simulink model "Landing_Gear_Simscape_multibody"  (R2026a)
settings: Solver=ode15s  StopTime=4.5  MaxStep=0.001  AbsTol=1e-3  EnableMultiTasking=on
libraries: sm_lib x42, nesl_utility x10, simulink x1
settings Model: Creator=USER  LastModifiedBy=USER
settings DebuggingCC: SubsystemReferenceDiagnosticForUnitTest=warning
settings SimscapeCC: SimscapeNominalValues="[{\"value\":\"1\",\"unit\":\"A\"},{\"value\":\"1\",\"unit\":\"bar\"},{\"value\":\"1\",\"unit\":\"cm^2\"},{\"value\":\"1\",\"unit\":\"cm^3/s\"},{\"value\":\"1\",\"unit\":\"kJ/kg\"},{\"value\":\"1\",\"unit\":\"kW\"},{\"value\":\"1\",\"unit\":\"l\"},{\"value\":\"1\",\"unit\":\"N\"},{\"value\":\"1\",\"unit\":\"N*m\"},{\"value\":\"1\",\"unit\":\"V\"}]"

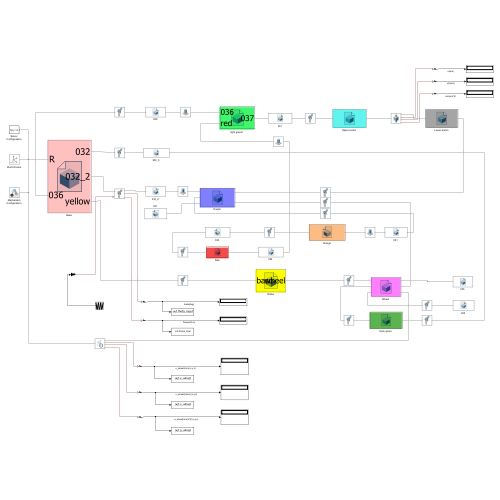
[thumbnail: Simulink's stored preview of the top-level diagram]
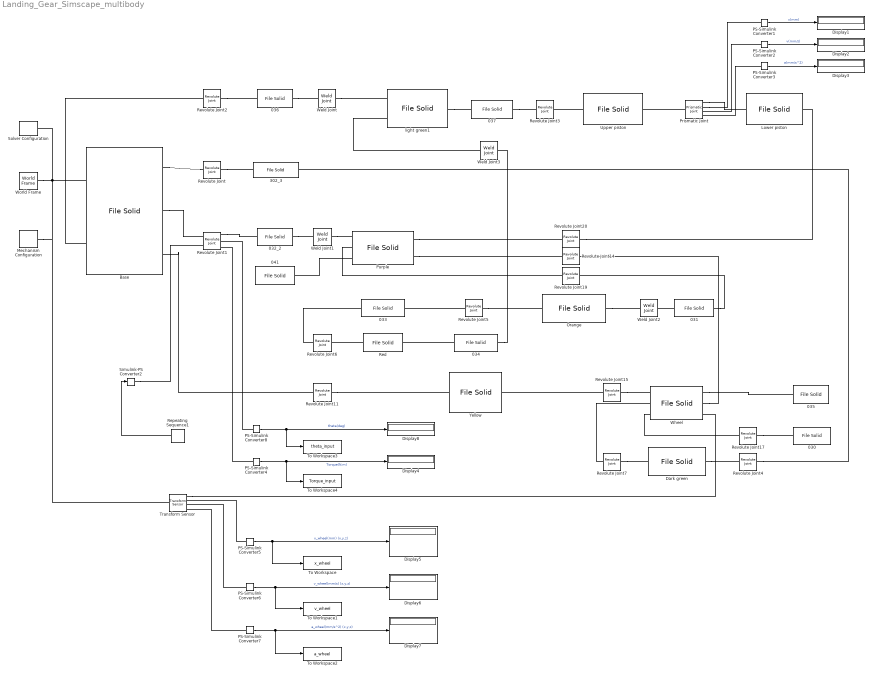
== system Landing_Gear_Simscape_multibody ==
  030 : sm_lib/Body Elements/File Solid  ExtGeomFileName=C:\Users\USER\Desktop\Term project Machinary\Term-Project-2103322-Design-of-Mechanism_Landing_Gear_Mechanism\simulation\cad\Parts\D0493-030.step  UnitType=FromFile  ExtGeomFileUnits=m  StepReaderType=HEX  ExportConvexHullGeometry=off  InertiaType=CalculateFromGeometry  BasedOnType=Density  Density=1000  DensityUnits=kg/m^3  Mass=1  MassUnits=kg  CenterOfMass=[0 0 0]  CenterOfMassUnits=m  MomentsOfInertia=[1 1 1]  MomentsOfInertiaUnits=kg*m^2  ProductsOfInertia=[0 0 0]  ProductsOfInertiaUnits=kg*m^2  GraphicType=FromGeometry  MarkerShape=Sphere  MarkerSize=10  GraphicVisPropType=FromFileVisualProperties  GraphicDiffuseColor=[0.5 0.5 0.5]  GraphicOpacity=1  GraphicSpecularColor=[0.5 0.5 0.5 1.0]  GraphicAmbientColor=[0.15 0.15 0.15 1.0]  GraphicEmissiveColor=[0.0 0.0 0.0 1.0]  GraphicShininess=75  DoExposeReferenceFrame=off  SerializedFrames=|
      | <Frames>
      | 
      |   <Frame>
      |     <Id>Frame1</Id>
      |     <Value>
      |       <Name>wheel</Name>
      |       <Origin>
      |         <Source>GeometricFeature</Source>
      |         <FeatureName>planar surface 2</FeatureName>
      |       </Origin>
      |       <PrimaryAxis>
      |         <DefinedDirection>+Z</DefinedDirection>
      |         <Source>ReferenceFrame</Source>
      |         <SourceDirection>+Z</SourceDirection>
      |         <FeatureName></FeatureName>
      |       </PrimaryAxis>
      |       <SecondaryAxis>
      |         <DefinedDirection>+X</DefinedDirection>
      |         <Source>ReferenceFrame</Source>
      |         <SourceDirection>+X</SourceDirection>
      |         <FeatureName></FeatureName>
      |       </SecondaryAxis>
      |     </Value>
      |   </Frame>
      | 
      | </Frames>
  031 : sm_lib/Body Elements/File Solid  ExtGeomFileName=C:\Users\USER\Desktop\Term project Machinary\Term-Project-2103322-Design-of-Mechanism_Landing_Gear_Mechanism\simulation\cad\Parts\D0493-031.step  UnitType=FromFile  ExtGeomFileUnits=m  StepReaderType=HEX  ExportConvexHullGeometry=off  InertiaType=CalculateFromGeometry  BasedOnType=Density  Density=1000  DensityUnits=kg/m^3  Mass=1  MassUnits=kg  CenterOfMass=[0 0 0]  CenterOfMassUnits=m  MomentsOfInertia=[1 1 1]  MomentsOfInertiaUnits=kg*m^2  ProductsOfInertia=[0 0 0]  ProductsOfInertiaUnits=kg*m^2  GraphicType=FromGeometry  MarkerShape=Sphere  MarkerSize=10  GraphicVisPropType=FromFileVisualProperties  GraphicDiffuseColor=[0.5 0.5 0.5]  GraphicOpacity=1  GraphicSpecularColor=[0.5 0.5 0.5 1.0]  GraphicAmbientColor=[0.15 0.15 0.15 1.0]  GraphicEmissiveColor=[0.0 0.0 0.0 1.0]  GraphicShininess=75  DoExposeReferenceFrame=off  SerializedFrames=|
      | <Frames>
      | 
      |   <Frame>
      |     <Id>Frame1</Id>
      |     <Value>
      |       <Name>orange</Name>
      |       <Origin>
      |         <Source>GeometricFeature</Source>
      |         <FeatureName>planar surface 1</FeatureName>
      |       </Origin>
      |       <PrimaryAxis>
      |         <DefinedDirection>+Z</DefinedDirection>
      |         <Source>ReferenceFrame</Source>
      |         <SourceDirection>+Z</SourceDirection>
      |         <FeatureName></FeatureName>
      |       </PrimaryAxis>
      |       <SecondaryAxis>
      |         <DefinedDirection>+X</DefinedDirection>
      |         <Source>ReferenceFrame</Source>
      |         <SourceDirection>+X</SourceDirection>
      |         <FeatureName></FeatureName>
      |       </SecondaryAxis>
      |     </Value>
      |   </Frame>
      | 
      |   <Frame>
      |     <Id>Frame2</Id>
      |     <Value>
      |       <Name>purple</Name>
      |       <Origin>
      |         <Source>GeometricFeature</Source>
      |         <FeatureName>cylindrical surface 2</FeatureName>
      |       </Origin>
      |       <PrimaryAxis>
      |         <DefinedDirection>+Z</DefinedDirection>
      |         <Source>ReferenceFrame</Source>
      |         <SourceDirection>+Z</SourceDirection>
      |         <FeatureName></FeatureName>
      |       </PrimaryAxis>
      |       <SecondaryAxis>
      |         <DefinedDirection>+X</DefinedDirection>
      |         <Source>ReferenceFrame</Source>
      |         <SourceDirection>+X</SourceDirection>
      |         <FeatureName></FeatureName>
      |       </SecondaryAxis>
      |     </Value>
      |   </Frame>
      | 
      | </Frames>
  032_2 : sm_lib/Body Elements/File Solid  ExtGeomFileName=C:\Users\USER\Desktop\Term project Machinary\Term-Project-2103322-Design-of-Mechanism_Landing_Gear_Mechanism\simulation\cad\Parts\D0493-032_2.step  UnitType=FromFile  ExtGeomFileUnits=m  StepReaderType=HEX  ExportConvexHullGeometry=off  InertiaType=CalculateFromGeometry  BasedOnType=Density  Density=1000  DensityUnits=kg/m^3  Mass=1  MassUnits=kg  CenterOfMass=[0 0 0]  CenterOfMassUnits=m  MomentsOfInertia=[1 1 1]  MomentsOfInertiaUnits=kg*m^2  ProductsOfInertia=[0 0 0]  ProductsOfInertiaUnits=kg*m^2  GraphicType=FromGeometry  MarkerShape=Sphere  MarkerSize=10  GraphicVisPropType=FromFileVisualProperties  GraphicDiffuseColor=[0.5 0.5 0.5]  GraphicOpacity=1  GraphicSpecularColor=[0.5 0.5 0.5 1.0]  GraphicAmbientColor=[0.15 0.15 0.15 1.0]  GraphicEmissiveColor=[0.0 0.0 0.0 1.0]  GraphicShininess=75  DoExposeReferenceFrame=off  SerializedFrames=|
      | <Frames>
      | 
      |   <Frame>
      |     <Id>Frame1</Id>
      |     <Value>
      |       <Name>base</Name>
      |       <Origin>
      |         <Source>GeometricFeature</Source>
      |         <FeatureName>planar surface 1</FeatureName>
      |       </Origin>
      |       <PrimaryAxis>
      |         <DefinedDirection>+Z</DefinedDirection>
      |         <Source>ReferenceFrame</Source>
      |         <SourceDirection>+Z</SourceDirection>
      |         <FeatureName></FeatureName>
      |       </PrimaryAxis>
      |       <SecondaryAxis>
      |         <DefinedDirection>+X</DefinedDirection>
      |         <Source>ReferenceFrame</Source>
      |         <SourceDirection>+X</SourceDirection>
      |         <FeatureName></FeatureName>
      |       </SecondaryAxis>
      |     </Value>
      |   </Frame>
      | 
      |   <Frame>
      |     <Id>Frame2</Id>
      |     <Value>
      |       <Name>purple</Name>
      |       <Origin>
      |         <Source>GeometricFeature</Source>
      |         <FeatureName>cylindrical surface 2</FeatureName>
      |       </Origin>
      |       <PrimaryAxis>
      |         <DefinedDirection>+Z</DefinedDirection>
      |         <Source>ReferenceFrame</Source>
      |         <SourceDirection>+Z</SourceDirection>
      |         <FeatureName></FeatureName>
      |       </PrimaryAxis>
      |       <SecondaryAxis>
      |         <DefinedDirection>+X</DefinedDirection>
      |         <Source>ReferenceFrame</Source>
      |         <SourceDirection>+X</SourceDirection>
      |         <FeatureName></FeatureName>
      |       </SecondaryAxis>
      |     </Value>
      |   </Frame>
      | 
      | </Frames>
  033 : sm_lib/Body Elements/File Solid  ExtGeomFileName=C:\Users\USER\Desktop\Term project Machinary\Term-Project-2103322-Design-of-Mechanism_Landing_Gear_Mechanism\simulation\cad\Parts\D0493-033.step  UnitType=FromFile  ExtGeomFileUnits=m  StepReaderType=HEX  ExportConvexHullGeometry=off  InertiaType=CalculateFromGeometry  BasedOnType=Density  Density=1000  DensityUnits=kg/m^3  Mass=1  MassUnits=kg  CenterOfMass=[0 0 0]  CenterOfMassUnits=m  MomentsOfInertia=[1 1 1]  MomentsOfInertiaUnits=kg*m^2  ProductsOfInertia=[0 0 0]  ProductsOfInertiaUnits=kg*m^2  GraphicType=FromGeometry  MarkerShape=Sphere  MarkerSize=10  GraphicVisPropType=FromFileVisualProperties  GraphicDiffuseColor=[0.5 0.5 0.5]  GraphicOpacity=1  GraphicSpecularColor=[0.5 0.5 0.5 1.0]  GraphicAmbientColor=[0.15 0.15 0.15 1.0]  GraphicEmissiveColor=[0.0 0.0 0.0 1.0]  GraphicShininess=75  DoExposeReferenceFrame=off  SerializedFrames=|
      | <Frames>
      | 
      |   <Frame>
      |     <Id>Frame1</Id>
      |     <Value>
      |       <Name>orange</Name>
      |       <Origin>
      |         <Source>GeometricFeature</Source>
      |         <FeatureName>planar surface 2</FeatureName>
      |       </Origin>
      |       <PrimaryAxis>
      |         <DefinedDirection>+Z</DefinedDirection>
      |         <Source>ReferenceFrame</Source>
      |         <SourceDirection>+Z</SourceDirection>
      |         <FeatureName></FeatureName>
      |       </PrimaryAxis>
      |       <SecondaryAxis>
      |         <DefinedDirection>+X</DefinedDirection>
      |         <Source>ReferenceFrame</Source>
      |         <SourceDirection>+X</SourceDirection>
      |         <FeatureName></FeatureName>
      |       </SecondaryAxis>
      |     </Value>
      |   </Frame>
      | 
      |   <Frame>
      |     <Id>Frame2</Id>
      |     <Value>
      |       <Name>red</Name>
      |       <Origin>
      |         <Source>GeometricFeature</Source>
      |         <FeatureName>cylindrical surface 2</FeatureName>
      |       </Origin>
      |       <PrimaryAxis>
      |         <DefinedDirection>+Z</DefinedDirection>
      |         <Source>ReferenceFrame</Source>
      |         <SourceDirection>+Z</SourceDirection>
      |         <FeatureName></FeatureName>
      |       </PrimaryAxis>
      |       <SecondaryAxis>
      |         <DefinedDirection>+X</DefinedDirection>
      |         <Source>ReferenceFrame</Source>
      |         <SourceDirection>+X</SourceDirection>
      |         <FeatureName></FeatureName>
      |       </SecondaryAxis>
      |     </Value>
      |   </Frame>
      | 
      | </Frames>
  034 : sm_lib/Body Elements/File Solid  ExtGeomFileName=C:\Users\USER\Desktop\Term project Machinary\Term-Project-2103322-Design-of-Mechanism_Landing_Gear_Mechanism\simulation\cad\Parts\D0493-034.step  UnitType=FromFile  ExtGeomFileUnits=m  StepReaderType=HEX  ExportConvexHullGeometry=off  InertiaType=CalculateFromGeometry  BasedOnType=Density  Density=1000  DensityUnits=kg/m^3  Mass=1  MassUnits=kg  CenterOfMass=[0 0 0]  CenterOfMassUnits=m  MomentsOfInertia=[1 1 1]  MomentsOfInertiaUnits=kg*m^2  ProductsOfInertia=[0 0 0]  ProductsOfInertiaUnits=kg*m^2  GraphicType=FromGeometry  MarkerShape=Sphere  MarkerSize=10  GraphicVisPropType=FromFileVisualProperties  GraphicDiffuseColor=[0.5 0.5 0.5]  GraphicOpacity=1  GraphicSpecularColor=[0.5 0.5 0.5 1.0]  GraphicAmbientColor=[0.15 0.15 0.15 1.0]  GraphicEmissiveColor=[0.0 0.0 0.0 1.0]  GraphicShininess=75  DoExposeReferenceFrame=off  SerializedFrames=|
      | <Frames>
      | 
      |   <Frame>
      |     <Id>Frame1</Id>
      |     <Value>
      |       <Name>red</Name>
      |       <Origin>
      |         <Source>GeometricFeature</Source>
      |         <FeatureName>planar surface 2</FeatureName>
      |       </Origin>
      |       <PrimaryAxis>
      |         <DefinedDirection>+Z</DefinedDirection>
      |         <Source>ReferenceFrame</Source>
      |         <SourceDirection>+Z</SourceDirection>
      |         <FeatureName></FeatureName>
      |       </PrimaryAxis>
      |       <SecondaryAxis>
      |         <DefinedDirection>+X</DefinedDirection>
      |         <Source>ReferenceFrame</Source>
      |         <SourceDirection>+X</SourceDirection>
      |         <FeatureName></FeatureName>
      |       </SecondaryAxis>
      |     </Value>
      |   </Frame>
      | 
      |   <Frame>
      |     <Id>Frame2</Id>
      |     <Value>
      |       <Name>lg</Name>
      |       <Origin>
      |         <Source>GeometricFeature</Source>
      |         <FeatureName>planar surface 2</FeatureName>
      |       </Origin>
      |       <PrimaryAxis>
      |         <DefinedDirection>+Z</DefinedDirection>
      |         <Source>ReferenceFrame</Source>
      |         <SourceDirection>+Z</SourceDirection>
      |         <FeatureName></FeatureName>
      |       </PrimaryAxis>
      |       <SecondaryAxis>
      |         <DefinedDirection>+X</DefinedDirection>
      |         <Source>ReferenceFrame</Source>
      |         <SourceDirection>+X</SourceDirection>
      |         <FeatureName></FeatureName>
      |       </SecondaryAxis>
      |     </Value>
      |   </Frame>
      | 
      | </Frames>
  035 : sm_lib/Body Elements/File Solid  ExtGeomFileName=C:\Users\USER\Desktop\Term project Machinary\Term-Project-2103322-Design-of-Mechanism_Landing_Gear_Mechanism\simulation\cad\Parts\D0493-035.step  UnitType=FromFile  ExtGeomFileUnits=m  StepReaderType=HEX  ExportConvexHullGeometry=off  InertiaType=CalculateFromGeometry  BasedOnType=Density  Density=1000  DensityUnits=kg/m^3  Mass=1  MassUnits=kg  CenterOfMass=[0 0 0]  CenterOfMassUnits=m  MomentsOfInertia=[1 1 1]  MomentsOfInertiaUnits=kg*m^2  ProductsOfInertia=[0 0 0]  ProductsOfInertiaUnits=kg*m^2  GraphicType=FromGeometry  MarkerShape=Sphere  MarkerSize=10  GraphicVisPropType=FromFileVisualProperties  GraphicDiffuseColor=[0.5 0.5 0.5]  GraphicOpacity=1  GraphicSpecularColor=[0.5 0.5 0.5 1.0]  GraphicAmbientColor=[0.15 0.15 0.15 1.0]  GraphicEmissiveColor=[0.0 0.0 0.0 1.0]  GraphicShininess=75  DoExposeReferenceFrame=off  SerializedFrames=|
      | <Frames>
      | 
      |   <Frame>
      |     <Id>Frame1</Id>
      |     <Value>
      |       <Name>wheel</Name>
      |       <Origin>
      |         <Source>GeometricFeature</Source>
      |         <FeatureName>planar surface 2</FeatureName>
      |       </Origin>
      |       <PrimaryAxis>
      |         <DefinedDirection>+Z</DefinedDirection>
      |         <Source>ReferenceFrame</Source>
      |         <SourceDirection>+Z</SourceDirection>
      |         <FeatureName></FeatureName>
      |       </PrimaryAxis>
      |       <SecondaryAxis>
      |         <DefinedDirection>+X</DefinedDirection>
      |         <Source>ReferenceFrame</Source>
      |         <SourceDirection>+X</SourceDirection>
      |         <FeatureName></FeatureName>
      |       </SecondaryAxis>
      |     </Value>
      |   </Frame>
      | 
      | </Frames>
  036 : sm_lib/Body Elements/File Solid  ExtGeomFileName=C:\Users\USER\Desktop\Term project Machinary\Term-Project-2103322-Design-of-Mechanism_Landing_Gear_Mechanism\simulation\cad\Parts\D0493-036.step  UnitType=FromFile  ExtGeomFileUnits=m  StepReaderType=HEX  ExportConvexHullGeometry=off  InertiaType=CalculateFromGeometry  BasedOnType=Density  Density=1000  DensityUnits=kg/m^3  Mass=1  MassUnits=kg  CenterOfMass=[0 0 0]  CenterOfMassUnits=m  MomentsOfInertia=[1 1 1]  MomentsOfInertiaUnits=kg*m^2  ProductsOfInertia=[0 0 0]  ProductsOfInertiaUnits=kg*m^2  GraphicType=FromGeometry  MarkerShape=Sphere  MarkerSize=10  GraphicVisPropType=FromFileVisualProperties  GraphicDiffuseColor=[0.5 0.5 0.5]  GraphicOpacity=1  GraphicSpecularColor=[0.5 0.5 0.5 1.0]  GraphicAmbientColor=[0.15 0.15 0.15 1.0]  GraphicEmissiveColor=[0.0 0.0 0.0 1.0]  GraphicShininess=75  DoExposeReferenceFrame=off  SerializedFrames=|
      | <Frames>
      | 
      |   <Frame>
      |     <Id>Frame1</Id>
      |     <Value>
      |       <Name>base</Name>
      |       <Origin>
      |         <Source>GeometricFeature</Source>
      |         <FeatureName>planar surface 2</FeatureName>
      |       </Origin>
      |       <PrimaryAxis>
      |         <DefinedDirection>+Z</DefinedDirection>
      |         <Source>ReferenceFrame</Source>
      |         <SourceDirection>+Z</SourceDirection>
      |         <FeatureName></FeatureName>
      |       </PrimaryAxis>
      |       <SecondaryAxis>
      |         <DefinedDirection>+X</DefinedDirection>
      |         <Source>ReferenceFrame</Source>
      |         <SourceDirection>+X</SourceDirection>
      |         <FeatureName></FeatureName>
      |       </SecondaryAxis>
      |     </Value>
      |   </Frame>
      | 
      |   <Frame>
      |     <Id>Frame2</Id>
      |     <Value>
      |       <Name>light g</Name>
      |       <Origin>
      |         <Source>GeometricFeature</Source>
      |         <FeatureName>cylindrical surface 2</FeatureName>
      |       </Origin>
      |       <PrimaryAxis>
      |         <DefinedDirection>+Z</DefinedDirection>
      |         <Source>ReferenceFrame</Source>
      |         <SourceDirection>+Z</SourceDirection>
      |         <FeatureName></FeatureName>
      |       </PrimaryAxis>
      |       <SecondaryAxis>
      |         <DefinedDirection>+X</DefinedDirection>
      |         <Source>ReferenceFrame</Source>
      |         <SourceDirection>+X</SourceDirection>
      |         <FeatureName></FeatureName>
      |       </SecondaryAxis>
      |     </Value>
      |   </Frame>
      | 
      | </Frames>
  037 : sm_lib/Body Elements/File Solid  ExtGeomFileName=C:\Users\USER\Desktop\Term project Machinary\Term-Project-2103322-Design-of-Mechanism_Landing_Gear_Mechanism\simulation\cad\Parts\D0493-037.step  UnitType=FromFile  ExtGeomFileUnits=m  StepReaderType=HEX  ExportConvexHullGeometry=off  InertiaType=CalculateFromGeometry  BasedOnType=Density  Density=1000  DensityUnits=kg/m^3  Mass=1  MassUnits=kg  CenterOfMass=[0 0 0]  CenterOfMassUnits=m  MomentsOfInertia=[1 1 1]  MomentsOfInertiaUnits=kg*m^2  ProductsOfInertia=[0 0 0]  ProductsOfInertiaUnits=kg*m^2  GraphicType=FromGeometry  MarkerShape=Sphere  MarkerSize=10  GraphicVisPropType=FromFileVisualProperties  GraphicDiffuseColor=[0.5 0.5 0.5]  GraphicOpacity=1  GraphicSpecularColor=[0.5 0.5 0.5 1.0]  GraphicAmbientColor=[0.15 0.15 0.15 1.0]  GraphicEmissiveColor=[0.0 0.0 0.0 1.0]  GraphicShininess=75  DoExposeReferenceFrame=off  SerializedFrames=|
      | <Frames>
      | 
      |   <Frame>
      |     <Id>Frame1</Id>
      |     <Value>
      |       <Name>light g</Name>
      |       <Origin>
      |         <Source>GeometricFeature</Source>
      |         <FeatureName>planar surface 1</FeatureName>
      |       </Origin>
      |       <PrimaryAxis>
      |         <DefinedDirection>+Z</DefinedDirection>
      |         <Source>ReferenceFrame</Source>
      |         <SourceDirection>+Z</SourceDirection>
      |         <FeatureName></FeatureName>
      |       </PrimaryAxis>
      |       <SecondaryAxis>
      |         <DefinedDirection>+X</DefinedDirection>
      |         <Source>ReferenceFrame</Source>
      |         <SourceDirection>+X</SourceDirection>
      |         <FeatureName></FeatureName>
      |       </SecondaryAxis>
      |     </Value>
      |   </Frame>
      | 
      |   <Frame>
      |     <Id>Frame2</Id>
      |     <Value>
      |       <Name>upper</Name>
      |       <Origin>
      |         <Source>GeometricFeature</Source>
      |         <FeatureName>circular curve 4</FeatureName>
      |       </Origin>
      |       <PrimaryAxis>
      |         <DefinedDirection>+Z</DefinedDirection>
      |         <Source>ReferenceFrame</Source>
      |         <SourceDirection>+Z</SourceDirection>
      |         <FeatureName></FeatureName>
      |       </PrimaryAxis>
      |       <SecondaryAxis>
      |         <DefinedDirection>+X</DefinedDirection>
      |         <Source>ReferenceFrame</Source>
      |         <SourceDirection>+X</SourceDirection>
      |         <FeatureName></FeatureName>
      |       </SecondaryAxis>
      |     </Value>
      |   </Frame>
      | 
      | </Frames>
  041 : sm_lib/Body Elements/File Solid  ExtGeomFileName=C:\Users\USER\Desktop\Term project Machinary\Term-Project-2103322-Design-of-Mechanism_Landing_Gear_Mechanism\simulation\cad\Parts\D0493-041.step  UnitType=FromFile  ExtGeomFileUnits=m  StepReaderType=HEX  ExportConvexHullGeometry=off  InertiaType=CalculateFromGeometry  BasedOnType=Density  Density=1000  DensityUnits=kg/m^3  Mass=1  MassUnits=kg  CenterOfMass=[0 0 0]  CenterOfMassUnits=m  MomentsOfInertia=[1 1 1]  MomentsOfInertiaUnits=kg*m^2  ProductsOfInertia=[0 0 0]  ProductsOfInertiaUnits=kg*m^2  GraphicType=FromGeometry  MarkerShape=Sphere  MarkerSize=10  GraphicVisPropType=FromFileVisualProperties  GraphicDiffuseColor=[0.5 0.5 0.5]  GraphicOpacity=1  GraphicSpecularColor=[0.5 0.5 0.5 1.0]  GraphicAmbientColor=[0.15 0.15 0.15 1.0]  GraphicEmissiveColor=[0.0 0.0 0.0 1.0]  GraphicShininess=75  DoExposeReferenceFrame=off  SerializedFrames=|
      | <Frames>
      | 
      |   <Frame>
      |     <Id>Frame1</Id>
      |     <Value>
      |       <Name>purple</Name>
      |       <Origin>
      |         <Source>GeometricFeature</Source>
      |         <FeatureName>planar surface 2</FeatureName>
      |       </Origin>
      |       <PrimaryAxis>
      |         <DefinedDirection>+Z</DefinedDirection>
      |         <Source>ReferenceFrame</Source>
      |         <SourceDirection>+Z</SourceDirection>
      |         <FeatureName></FeatureName>
      |       </PrimaryAxis>
      |       <SecondaryAxis>
      |         <DefinedDirection>+X</DefinedDirection>
      |         <Source>ReferenceFrame</Source>
      |         <SourceDirection>+X</SourceDirection>
      |         <FeatureName></FeatureName>
      |       </SecondaryAxis>
      |     </Value>
      |   </Frame>
      | 
      | </Frames>
  302_3 : sm_lib/Body Elements/File Solid  ExtGeomFileName=C:\Users\USER\Desktop\Term project Machinary\Term-Project-2103322-Design-of-Mechanism_Landing_Gear_Mechanism\simulation\cad\Parts\D0493-032_3.step  UnitType=FromFile  ExtGeomFileUnits=m  StepReaderType=HEX  ExportConvexHullGeometry=off  InertiaType=CalculateFromGeometry  BasedOnType=Density  Density=1000  DensityUnits=kg/m^3  Mass=1  MassUnits=kg  CenterOfMass=[0 0 0]  CenterOfMassUnits=m  MomentsOfInertia=[1 1 1]  MomentsOfInertiaUnits=kg*m^2  ProductsOfInertia=[0 0 0]  ProductsOfInertiaUnits=kg*m^2  GraphicType=FromGeometry  MarkerShape=Sphere  MarkerSize=10  GraphicVisPropType=FromFileVisualProperties  GraphicDiffuseColor=[0.5 0.5 0.5]  GraphicOpacity=1  GraphicSpecularColor=[0.5 0.5 0.5 1.0]  GraphicAmbientColor=[0.15 0.15 0.15 1.0]  GraphicEmissiveColor=[0.0 0.0 0.0 1.0]  GraphicShininess=75  DoExposeReferenceFrame=off  SerializedFrames=|
      | <Frames>
      | 
      |   <Frame>
      |     <Id>Frame1</Id>
      |     <Value>
      |       <Name>Base</Name>
      |       <Origin>
      |         <Source>GeometricFeature</Source>
      |         <FeatureName>planar surface 1</FeatureName>
      |       </Origin>
      |       <PrimaryAxis>
      |         <DefinedDirection>+Z</DefinedDirection>
      |         <Source>ReferenceFrame</Source>
      |         <SourceDirection>+Z</SourceDirection>
      |         <FeatureName></FeatureName>
      |       </PrimaryAxis>
      |       <SecondaryAxis>
      |         <DefinedDirection>+X</DefinedDirection>
      |         <Source>ReferenceFrame</Source>
      |         <SourceDirection>+X</SourceDirection>
      |         <FeatureName></FeatureName>
      |       </SecondaryAxis>
      |     </Value>
      |   </Frame>
      | 
      |   <Frame>
      |     <Id>Frame2</Id>
      |     <Value>
      |       <Name>darkgreen</Name>
      |       <Origin>
      |         <Source>GeometricFeature</Source>
      |         <FeatureName>cylindrical surface 1</FeatureName>
      |       </Origin>
      |       <PrimaryAxis>
      |         <DefinedDirection>+Z</DefinedDirection>
      |         <Source>ReferenceFrame</Source>
      |         <SourceDirection>+Z</SourceDirection>
      |         <FeatureName></FeatureName>
      |       </PrimaryAxis>
      |       <SecondaryAxis>
      |         <DefinedDirection>+X</DefinedDirection>
      |         <Source>ReferenceFrame</Source>
      |         <SourceDirection>+X</SourceDirection>
      |         <FeatureName></FeatureName>
      |       </SecondaryAxis>
      |     </Value>
      |   </Frame>
      | 
      | </Frames>
  Base : sm_lib/Body Elements/File Solid  ExtGeomFileName=C:\Users\USER\Desktop\Term project Machinary\Term-Project-2103322-Design-of-Mechanism_Landing_Gear_Mechanism\simulation\cad\Parts\Base.step  UnitType=FromFile  ExtGeomFileUnits=m  StepReaderType=HEX  ExportConvexHullGeometry=off  InertiaType=CalculateFromGeometry  BasedOnType=Density  Density=1000  DensityUnits=kg/m^3  Mass=1  MassUnits=kg  CenterOfMass=[0 0 0]  CenterOfMassUnits=m  MomentsOfInertia=[1 1 1]  MomentsOfInertiaUnits=kg*m^2  ProductsOfInertia=[0 0 0]  ProductsOfInertiaUnits=kg*m^2  GraphicType=FromGeometry  MarkerShape=Sphere  MarkerSize=10  GraphicVisPropType=FromFileVisualProperties  GraphicDiffuseColor=[0.5 0.5 0.5]  GraphicOpacity=1  GraphicSpecularColor=[0.5 0.5 0.5 1.0]  GraphicAmbientColor=[0.15 0.15 0.15 1.0]  GraphicEmissiveColor=[0.0 0.0 0.0 1.0]  GraphicShininess=75  DoExposeReferenceFrame=on  SerializedFrames=|
      | <Frames>
      | 
      |   <Frame>
      |     <Id>Frame1</Id>
      |     <Value>
      |       <Name>032</Name>
      |       <Origin>
      |         <Source>GeometricFeature</Source>
      |         <FeatureName>circular curve 21</FeatureName>
      |       </Origin>
      |       <PrimaryAxis>
      |         <DefinedDirection>+Z</DefinedDirection>
      |         <Source>GeometricFeature</Source>
      |         <SourceDirection>+Z</SourceDirection>
      |         <FeatureName>circular curve 33</FeatureName>
      |       </PrimaryAxis>
      |       <SecondaryAxis>
      |         <DefinedDirection>+Y</DefinedDirection>
      |         <Source>ReferenceFrame</Source>
      |         <SourceDirection>+Y</SourceDirection>
      |         <FeatureName></FeatureName>
      |       </SecondaryAxis>
      |     </Value>
      |   </Frame>
      | 
      |   <Frame>
      |     <Id>Frame2</Id>
      |     <Value>
      |       <Name>032_2</Name>
      |       <Origin>
      |         <Source>GeometricFeature</Source>
      |         <FeatureName>circular curve 35</FeatureName>
      |       </Origin>
      |       <PrimaryAxis>
      |         <DefinedDirection>+Z</DefinedDirection>
      |         <Source>GeometricFeature</Source>
      |         <SourceDirection>+Z</SourceDirection>
      |         <FeatureName>circular curve 35</FeatureName>
      |       </PrimaryAxis>
      |       <SecondaryAxis>
      |         <DefinedDirection>+Y</DefinedDirection>
      |         <Source>ReferenceFrame</Source>
      |         <SourceDirection>+Y</SourceDirection>
      |         <FeatureName></FeatureName>
      |       </SecondaryAxis>
      |     </Value>
      |   </Frame>
      | 
      |   <Frame>
      |     <Id>Frame3</Id>
      |     <Value>
      |       <Name>036</Name>
      |       <Origin>
      |         <Source>GeometricFeature</Source>
      |         <FeatureName>circular curve 89</FeatureName>
      |       </Origin>
      |       <PrimaryAxis>
      |         <DefinedDirection>-Z</DefinedDirection>
      |         <Source>GeometricFeature</Source>
      |         <SourceDirection>+Z</SourceDirection>
      |         <FeatureName>circular curve 89</FeatureName>
      |       </PrimaryAxis>
      |       <SecondaryAxis>
      |         <DefinedDirection>+Y</DefinedDirection>
      |         <Source>ReferenceFrame</Source>
      |         <SourceDirection>+Y</SourceDirection>
      |         <FeatureName></FeatureName>
      |       </SecondaryAxis>
      |     </Value>
      |   </Frame>
      | 
      |   <Frame>
      |     <Id>Frame4</Id>
      |     <Value>
      |       <Name>yellow</Name>
      |       <Origin>
      |         <Source>GeometricFeature</Source>
      |         <FeatureName>circular curve 60</FeatureName>
      |       </Origin>
      |       <PrimaryAxis>
      |         <DefinedDirection>+Z</DefinedDirection>
      |         <Source>GeometricFeature</Source>
      |         <SourceDirection>+Z</SourceDirection>
      |         <FeatureName>circular curve 60</FeatureName>
      |       </PrimaryAxis>
      |       <SecondaryAxis>
      |         <DefinedDirection>+Y</DefinedDirection>
      |         <Source>ReferenceFrame</Source>
      |         <SourceDirection>+Y</SourceDirection>
      |         <FeatureName></FeatureName>
      |       </SecondaryAxis>
      |     </Value>
      |   </Frame>
      | 
      | </Frames>
  Dark green : sm_lib/Body Elements/File Solid  ExtGeomFileName=C:\Users\USER\Desktop\Term project Machinary\Term-Project-2103322-Design-of-Mechanism_Landing_Gear_Mechanism\simulation\cad\Parts\Dark green.step  UnitType=FromFile  ExtGeomFileUnits=m  StepReaderType=HEX  ExportConvexHullGeometry=off  InertiaType=CalculateFromGeometry  BasedOnType=Density  Density=1000  DensityUnits=kg/m^3  Mass=1  MassUnits=kg  CenterOfMass=[0 0 0]  CenterOfMassUnits=m  MomentsOfInertia=[1 1 1]  MomentsOfInertiaUnits=kg*m^2  ProductsOfInertia=[0 0 0]  ProductsOfInertiaUnits=kg*m^2  GraphicType=FromGeometry  MarkerShape=Sphere  MarkerSize=10  GraphicVisPropType=FromFileVisualProperties  GraphicDiffuseColor=[0.5 0.5 0.5]  GraphicOpacity=1  GraphicSpecularColor=[0.5 0.5 0.5 1.0]  GraphicAmbientColor=[0.15 0.15 0.15 1.0]  GraphicEmissiveColor=[0.0 0.0 0.0 1.0]  GraphicShininess=75  DoExposeReferenceFrame=off  SerializedFrames=|
      | <Frames>
      | 
      |   <Frame>
      |     <Id>Frame1</Id>
      |     <Value>
      |       <Name>wheel</Name>
      |       <Origin>
      |         <Source>GeometricFeature</Source>
      |         <FeatureName>circular curve 51</FeatureName>
      |       </Origin>
      |       <PrimaryAxis>
      |         <DefinedDirection>+Z</DefinedDirection>
      |         <Source>GeometricFeature</Source>
      |         <SourceDirection>+Z</SourceDirection>
      |         <FeatureName>circular curve 51</FeatureName>
      |       </PrimaryAxis>
      |       <SecondaryAxis>
      |         <DefinedDirection>+Y</DefinedDirection>
      |         <Source>ReferenceFrame</Source>
      |         <SourceDirection>+Y</SourceDirection>
      |         <FeatureName></FeatureName>
      |       </SecondaryAxis>
      |     </Value>
      |   </Frame>
      | 
      |   <Frame>
      |     <Id>Frame2</Id>
      |     <Value>
      |       <Name>base</Name>
      |       <Origin>
      |         <Source>GeometricFeature</Source>
      |         <FeatureName>cylindrical surface 10</FeatureName>
      |       </Origin>
      |       <PrimaryAxis>
      |         <DefinedDirection>+Z</DefinedDirection>
      |         <Source>GeometricFeature</Source>
      |         <SourceDirection>+Z</SourceDirection>
      |         <FeatureName>cylindrical surface 10</FeatureName>
      |       </PrimaryAxis>
      |       <SecondaryAxis>
      |         <DefinedDirection>+Y</DefinedDirection>
      |         <Source>ReferenceFrame</Source>
      |         <SourceDirection>+Y</SourceDirection>
      |         <FeatureName></FeatureName>
      |       </SecondaryAxis>
      |     </Value>
      |   </Frame>
      | 
      | </Frames>
  Display{1..8} (8 alike) : Display
  Lower piston : sm_lib/Body Elements/File Solid  ExtGeomFileName=C:\Users\USER\Desktop\Term project Machinary\Term-Project-2103322-Design-of-Mechanism_Landing_Gear_Mechanism\simulation\cad\Parts\Lower_Piston2.step  UnitType=FromFile  ExtGeomFileUnits=m  StepReaderType=HEX  ExportConvexHullGeometry=off  InertiaType=CalculateFromGeometry  BasedOnType=Density  Density=1000  DensityUnits=kg/m^3  Mass=1  MassUnits=kg  CenterOfMass=[0 0 0]  CenterOfMassUnits=m  MomentsOfInertia=[1 1 1]  MomentsOfInertiaUnits=kg*m^2  ProductsOfInertia=[0 0 0]  ProductsOfInertiaUnits=kg*m^2  GraphicType=FromGeometry  MarkerShape=Sphere  MarkerSize=10  GraphicVisPropType=FromFileVisualProperties  GraphicDiffuseColor=[0.5 0.5 0.5]  GraphicOpacity=1  GraphicSpecularColor=[0.5 0.5 0.5 1.0]  GraphicAmbientColor=[0.15 0.15 0.15 1.0]  GraphicEmissiveColor=[0.0 0.0 0.0 1.0]  GraphicShininess=75  DoExposeReferenceFrame=off  SerializedFrames=|
      | <Frames>
      | 
      |   <Frame>
      |     <Id>Frame1</Id>
      |     <Value>
      |       <Name>upper</Name>
      |       <Origin>
      |         <Source>GeometricFeature</Source>
      |         <FeatureName>circular curve 40</FeatureName>
      |       </Origin>
      |       <PrimaryAxis>
      |         <DefinedDirection>-Z</DefinedDirection>
      |         <Source>GeometricFeature</Source>
      |         <SourceDirection>+Z</SourceDirection>
      |         <FeatureName>circular curve 40</FeatureName>
      |       </PrimaryAxis>
      |       <SecondaryAxis>
      |         <DefinedDirection>+X</DefinedDirection>
      |         <Source>ReferenceFrame</Source>
      |         <SourceDirection>+X</SourceDirection>
      |         <FeatureName></FeatureName>
      |       </SecondaryAxis>
      |     </Value>
      |   </Frame>
      | 
      |   <Frame>
      |     <Id>Frame2</Id>
      |     <Value>
      |       <Name>purple</Name>
      |       <Origin>
      |         <Source>GeometricFeature</Source>
      |         <FeatureName>circular curve 37</FeatureName>
      |       </Origin>
      |       <PrimaryAxis>
      |         <DefinedDirection>+Z</DefinedDirection>
      |         <Source>GeometricFeature</Source>
      |         <SourceDirection>+Z</SourceDirection>
      |         <FeatureName>circular curve 37</FeatureName>
      |       </PrimaryAxis>
      |       <SecondaryAxis>
      |         <DefinedDirection>+Y</DefinedDirection>
      |         <Source>ReferenceFrame</Source>
      |         <SourceDirection>+Y</SourceDirection>
      |         <FeatureName></FeatureName>
      |       </SecondaryAxis>
      |     </Value>
      |   </Frame>
      | 
      | </Frames>
  Mechanism Configuration : sm_lib/Utilities/Mechanism Configuration  UniformGravity=Constant  GravityVector=[0 0 -9.80665]  GravityVectorUnits=m/s^2  LinearizationDelta=0.001  JointModeTransitionNonlinearIterations=2
  Orange : sm_lib/Body Elements/File Solid  ExtGeomFileName=C:\Users\USER\Desktop\Term project Machinary\Term-Project-2103322-Design-of-Mechanism_Landing_Gear_Mechanism\simulation\cad\Parts\Orange.step  UnitType=FromFile  ExtGeomFileUnits=m  StepReaderType=HEX  ExportConvexHullGeometry=off  InertiaType=CalculateFromGeometry  BasedOnType=Density  Density=1000  DensityUnits=kg/m^3  Mass=1  MassUnits=kg  CenterOfMass=[0 0 0]  CenterOfMassUnits=m  MomentsOfInertia=[1 1 1]  MomentsOfInertiaUnits=kg*m^2  ProductsOfInertia=[0 0 0]  ProductsOfInertiaUnits=kg*m^2  GraphicType=FromGeometry  MarkerShape=Sphere  MarkerSize=10  GraphicVisPropType=FromFileVisualProperties  GraphicDiffuseColor=[0.5 0.5 0.5]  GraphicOpacity=1  GraphicSpecularColor=[0.5 0.5 0.5 1.0]  GraphicAmbientColor=[0.15 0.15 0.15 1.0]  GraphicEmissiveColor=[0.0 0.0 0.0 1.0]  GraphicShininess=75  DoExposeReferenceFrame=off  SerializedFrames=|
      | <Frames>
      | 
      |   <Frame>
      |     <Id>Frame1</Id>
      |     <Value>
      |       <Name>031</Name>
      |       <Origin>
      |         <Source>GeometricFeature</Source>
      |         <FeatureName>circular curve 22</FeatureName>
      |       </Origin>
      |       <PrimaryAxis>
      |         <DefinedDirection>-Z</DefinedDirection>
      |         <Source>GeometricFeature</Source>
      |         <SourceDirection>+Z</SourceDirection>
      |         <FeatureName>circular curve 22</FeatureName>
      |       </PrimaryAxis>
      |       <SecondaryAxis>
      |         <DefinedDirection>+Y</DefinedDirection>
      |         <Source>ReferenceFrame</Source>
      |         <SourceDirection>+Y</SourceDirection>
      |         <FeatureName></FeatureName>
      |       </SecondaryAxis>
      |     </Value>
      |   </Frame>
      | 
      |   <Frame>
      |     <Id>Frame2</Id>
      |     <Value>
      |       <Name>033</Name>
      |       <Origin>
      |         <Source>GeometricFeature</Source>
      |         <FeatureName>circular curve 58</FeatureName>
      |       </Origin>
      |       <PrimaryAxis>
      |         <DefinedDirection>-Z</DefinedDirection>
      |         <Source>GeometricFeature</Source>
      |         <SourceDirection>+Z</SourceDirection>
      |         <FeatureName>circular curve 58</FeatureName>
      |       </PrimaryAxis>
      |       <SecondaryAxis>
      |         <DefinedDirection>+Y</DefinedDirection>
      |         <Source>ReferenceFrame</Source>
      |         <SourceDirection>+Y</SourceDirection>
      |         <FeatureName></FeatureName>
      |       </SecondaryAxis>
      |     </Value>
      |   </Frame>
      | 
      | </Frames>
  PS-Simulink Converter1 : nesl_utility/PS-Simulink Converter  PhysicalDomain=network_engine_domain  SubClassName=ps_output  LeftPortType=input  RightPortType=output  PseudoPeriodic=off  Frequencies=[]  VectorFormat=inherit  Unit=mm  AffineConversion=off
  PS-Simulink Converter2 : nesl_utility/PS-Simulink Converter  PhysicalDomain=network_engine_domain  SubClassName=ps_output  LeftPortType=input  RightPortType=output  PseudoPeriodic=off  Frequencies=[]  VectorFormat=inherit  Unit=mm/s  AffineConversion=off
  PS-Simulink Converter3 : nesl_utility/PS-Simulink Converter  PhysicalDomain=network_engine_domain  SubClassName=ps_output  LeftPortType=input  RightPortType=output  PseudoPeriodic=off  Frequencies=[]  VectorFormat=inherit  Unit=mm/s^2  AffineConversion=off
  PS-Simulink Converter4 : nesl_utility/PS-Simulink Converter  PhysicalDomain=network_engine_domain  SubClassName=ps_output  LeftPortType=input  RightPortType=output  PseudoPeriodic=off  Frequencies=[]  VectorFormat=1-D array  Unit=N*m  AffineConversion=off
  PS-Simulink Converter5 : nesl_utility/PS-Simulink Converter  PhysicalDomain=network_engine_domain  SubClassName=ps_output  LeftPortType=input  RightPortType=output  PseudoPeriodic=off  Frequencies=[]  VectorFormat=inherit  Unit=mm  AffineConversion=off
  PS-Simulink Converter6 : nesl_utility/PS-Simulink Converter  PhysicalDomain=network_engine_domain  SubClassName=ps_output  LeftPortType=input  RightPortType=output  PseudoPeriodic=off  Frequencies=[]  VectorFormat=inherit  Unit=mm/s  AffineConversion=off
  PS-Simulink Converter7 : nesl_utility/PS-Simulink Converter  PhysicalDomain=network_engine_domain  SubClassName=ps_output  LeftPortType=input  RightPortType=output  PseudoPeriodic=off  Frequencies=[]  VectorFormat=inherit  Unit=mm/s^2  AffineConversion=off
  PS-Simulink Converter8 : nesl_utility/PS-Simulink Converter  PhysicalDomain=network_engine_domain  SubClassName=ps_output  LeftPortType=input  RightPortType=output  PseudoPeriodic=off  Frequencies=[]  VectorFormat=1-D array  Unit=deg  AffineConversion=off
  Prismatic Joint : sm_lib/Joints/Prismatic Joint  JointMode=Normal  CompositeWrenchDir=FollowerOnBase  CompositeWrenchFrame=BaseFrame  SenseConstraintForce=off  SenseConstraintTorque=off  SenseTotalForce=off  SenseTotalTorque=off  PositionTargetSpecify=off  PositionTargetPriority=High  PositionTargetValue=0  PositionTargetValueUnits=m  VelocityTargetSpecify=off  VelocityTargetPriority=High  VelocityTargetValue=0  VelocityTargetValueUnits=m/s  EquilibriumPosition=0  EquilibriumPositionUnits=m  SpringStiffness=0  SpringStiffnessUnits=N/m  DampingCoefficient=0  DampingCoefficientUnits=N/(m/s)  LowerLimitSpecify=off  LowerLimitBound=-1  LowerLimitBoundUnits=m  LowerLimitStiffness=1e6  LowerLimitStiffnessUnits=N/m  LowerLimitDamping=1e3  LowerLimitDampingUnits=N/(m/s)  LowerLimitTransitionRegionWidth=1e-4  LowerLimitTransitionRegionWidthUnits=m  UpperLimitSpecify=off  UpperLimitBound=1  UpperLimitBoundUnits=m  UpperLimitStiffness=1e6  UpperLimitStiffnessUnits=N/m  UpperLimitDamping=1e3  UpperLimitDampingUnits=N/(m/s)  UpperLimitTransitionRegionWidth=1e-4  UpperLimitTransitionRegionWidthUnits=m  TorqueActuationMode=NoTorque  MotionActuationMode=ComputedMotion  SensePosition=on  SenseVelocity=on  SenseAcceleration=on  SenseTorqueForce=off  SenseLowerLimitTorqueForce=off  SenseUpperLimitTorqueForce=off
  Purple : sm_lib/Body Elements/File Solid  ExtGeomFileName=C:\Users\USER\Desktop\Term project Machinary\Term-Project-2103322-Design-of-Mechanism_Landing_Gear_Mechanism\simulation\cad\Parts\Purple.step  UnitType=FromFile  ExtGeomFileUnits=m  StepReaderType=HEX  ExportConvexHullGeometry=off  InertiaType=CalculateFromGeometry  BasedOnType=Density  Density=1000  DensityUnits=kg/m^3  Mass=1  MassUnits=kg  CenterOfMass=[0 0 0]  CenterOfMassUnits=m  MomentsOfInertia=[1 1 1]  MomentsOfInertiaUnits=kg*m^2  ProductsOfInertia=[0 0 0]  ProductsOfInertiaUnits=kg*m^2  GraphicType=FromGeometry  MarkerShape=Sphere  MarkerSize=10  GraphicVisPropType=FromFileVisualProperties  GraphicDiffuseColor=[0.5 0.5 0.5]  GraphicOpacity=1  GraphicSpecularColor=[0.5 0.5 0.5 1.0]  GraphicAmbientColor=[0.15 0.15 0.15 1.0]  GraphicEmissiveColor=[0.0 0.0 0.0 1.0]  GraphicShininess=75  DoExposeReferenceFrame=off  SerializedFrames=|
      | <Frames>
      | 
      |   <Frame>
      |     <Id>Frame1</Id>
      |     <Value>
      |       <Name>base</Name>
      |       <Origin>
      |         <Source>GeometricFeature</Source>
      |         <FeatureName>cylindrical surface 21</FeatureName>
      |       </Origin>
      |       <PrimaryAxis>
      |         <DefinedDirection>+Z</DefinedDirection>
      |         <Source>GeometricFeature</Source>
      |         <SourceDirection>+Z</SourceDirection>
      |         <FeatureName>cylindrical surface 21</FeatureName>
      |       </PrimaryAxis>
      |       <SecondaryAxis>
      |         <DefinedDirection>+Y</DefinedDirection>
      |         <Source>ReferenceFrame</Source>
      |         <SourceDirection>+Y</SourceDirection>
      |         <FeatureName></FeatureName>
      |       </SecondaryAxis>
      |     </Value>
      |   </Frame>
      | 
      |   <Frame>
      |     <Id>Frame2</Id>
      |     <Value>
      |       <Name>lower</Name>
      |       <Origin>
      |         <Source>GeometricFeature</Source>
      |         <FeatureName>circular curve 37</FeatureName>
      |       </Origin>
      |       <PrimaryAxis>
      |         <DefinedDirection>-Z</DefinedDirection>
      |         <Source>GeometricFeature</Source>
      |         <SourceDirection>+Z</SourceDirection>
      |         <FeatureName>circular curve 37</FeatureName>
      |       </PrimaryAxis>
      |       <SecondaryAxis>
      |         <DefinedDirection>+Y</DefinedDirection>
      |         <Source>ReferenceFrame</Source>
      |         <SourceDirection>+Y</SourceDirection>
      |         <FeatureName></FeatureName>
      |       </SecondaryAxis>
      |     </Value>
      |   </Frame>
      | 
      |   <Frame>
      |     <Id>Frame3</Id>
      |     <Value>
      |       <Name>orange</Name>
      |       <Origin>
      |         <Source>GeometricFeature</Source>
      |         <FeatureName>cylindrical surface 33</FeatureName>
      |       </Origin>
      |       <PrimaryAxis>
      |         <DefinedDirection>+Z</DefinedDirection>
      |         <Source>GeometricFeature</Source>
      |         <SourceDirection>+Z</SourceDirection>
      |         <FeatureName>cylindrical surface 33</FeatureName>
      |       </PrimaryAxis>
      |       <SecondaryAxis>
      |         <DefinedDirection>+Y</DefinedDirection>
      |         <Source>ReferenceFrame</Source>
      |         <SourceDirection>+Y</SourceDirection>
      |         <FeatureName></FeatureName>
      |       </SecondaryAxis>
      |     </Value>
      |   </Frame>
      | 
      |   <Frame>
      |     <Id>Frame4</Id>
      |     <Value>
      |       <Name>wheel</Name>
      |       <Origin>
      |         <Source>GeometricFeature</Source>
      |         <FeatureName>circular curve 82</FeatureName>
      |       </Origin>
      |       <PrimaryAxis>
      |         <DefinedDirection>+Z</DefinedDirection>
      |         <Source>GeometricFeature</Source>
      |         <SourceDirection>+Z</SourceDirection>
      |         <FeatureName>circular curve 95</FeatureName>
      |       </PrimaryAxis>
      |       <SecondaryAxis>
      |         <DefinedDirection>+Y</DefinedDirection>
      |         <Source>ReferenceFrame</Source>
      |         <SourceDirection>+Y</SourceDirection>
      |         <FeatureName></FeatureName>
      |       </SecondaryAxis>
      |     </Value>
      |   </Frame>
      | 
      |   <Frame>
      |     <Id>Frame5</Id>
      |     <Value>
      |       <Name>041</Name>
      |       <Origin>
      |         <Source>GeometricFeature</Source>
      |         <FeatureName>circular curve 29</FeatureName>
      |       </Origin>
      |       <PrimaryAxis>
      |         <DefinedDirection>+Z</DefinedDirection>
      |         <Source>GeometricFeature</Source>
      |         <SourceDirection>+Z</SourceDirection>
      |         <FeatureName>circular curve 29</FeatureName>
      |       </PrimaryAxis>
      |       <SecondaryAxis>
      |         <DefinedDirection>+Y</DefinedDirection>
      |         <Source>ReferenceFrame</Source>
      |         <SourceDirection>+Y</SourceDirection>
      |         <FeatureName></FeatureName>
      |       </SecondaryAxis>
      |     </Value>
      |   </Frame>
      | 
      | </Frames>
  Red : sm_lib/Body Elements/File Solid  ExtGeomFileName=C:\Users\USER\Desktop\Term project Machinary\Term-Project-2103322-Design-of-Mechanism_Landing_Gear_Mechanism\simulation\cad\Parts\Red.step  UnitType=FromFile  ExtGeomFileUnits=m  StepReaderType=HEX  ExportConvexHullGeometry=off  InertiaType=CalculateFromGeometry  BasedOnType=Density  Density=1000  DensityUnits=kg/m^3  Mass=1  MassUnits=kg  CenterOfMass=[0 0 0]  CenterOfMassUnits=m  MomentsOfInertia=[1 1 1]  MomentsOfInertiaUnits=kg*m^2  ProductsOfInertia=[0 0 0]  ProductsOfInertiaUnits=kg*m^2  GraphicType=FromGeometry  MarkerShape=Sphere  MarkerSize=10  GraphicVisPropType=FromFileVisualProperties  GraphicDiffuseColor=[0.5 0.5 0.5]  GraphicOpacity=1  GraphicSpecularColor=[0.5 0.5 0.5 1.0]  GraphicAmbientColor=[0.15 0.15 0.15 1.0]  GraphicEmissiveColor=[0.0 0.0 0.0 1.0]  GraphicShininess=75  DoExposeReferenceFrame=off  SerializedFrames=|
      | <Frames>
      | 
      |   <Frame>
      |     <Id>Frame1</Id>
      |     <Value>
      |       <Name>033</Name>
      |       <Origin>
      |         <Source>GeometricFeature</Source>
      |         <FeatureName>cylindrical surface 13</FeatureName>
      |       </Origin>
      |       <PrimaryAxis>
      |         <DefinedDirection>-Z</DefinedDirection>
      |         <Source>GeometricFeature</Source>
      |         <SourceDirection>+Z</SourceDirection>
      |         <FeatureName>cylindrical surface 13</FeatureName>
      |       </PrimaryAxis>
      |       <SecondaryAxis>
      |         <DefinedDirection>+Y</DefinedDirection>
      |         <Source>ReferenceFrame</Source>
      |         <SourceDirection>+Y</SourceDirection>
      |         <FeatureName></FeatureName>
      |       </SecondaryAxis>
      |     </Value>
      |   </Frame>
      | 
      |   <Frame>
      |     <Id>Frame2</Id>
      |     <Value>
      |       <Name>034</Name>
      |       <Origin>
      |         <Source>GeometricFeature</Source>
      |         <FeatureName>circular curve 4</FeatureName>
      |       </Origin>
      |       <PrimaryAxis>
      |         <DefinedDirection>+Z</DefinedDirection>
      |         <Source>GeometricFeature</Source>
      |         <SourceDirection>+Z</SourceDirection>
      |         <FeatureName>circular curve 4</FeatureName>
      |       </PrimaryAxis>
      |       <SecondaryAxis>
      |         <DefinedDirection>+X</DefinedDirection>
      |         <Source>ReferenceFrame</Source>
      |         <SourceDirection>+X</SourceDirection>
      |         <FeatureName></FeatureName>
      |       </SecondaryAxis>
      |     </Value>
      |   </Frame>
      | 
      | </Frames>
  Repeating Sequence1 : simulink/Sources/Repeating Sequence  rep_seq_t=[0 4.5 6 12]  rep_seq_y=[-0.11454782472119 -1.7280948939871 -1.7280948939871 -0.11454782472119]
  Revolute Joint{,2..7,14..15,17,19} (11 alike) : sm_lib/Joints/Revolute Joint  JointMode=Normal  CompositeWrenchDir=FollowerOnBase  CompositeWrenchFrame=BaseFrame  SenseConstraintForce=off  SenseConstraintTorque=off  SenseTotalForce=off  SenseTotalTorque=off  PositionTargetSpecify=off  PositionTargetPriority=High  PositionTargetValue=0  PositionTargetValueUnits=deg  VelocityTargetSpecify=off  VelocityTargetPriority=High  VelocityTargetValue=0  VelocityTargetValueUnits=deg/s  EquilibriumPosition=0  EquilibriumPositionUnits=deg  SpringStiffness=0  SpringStiffnessUnits=N*m/deg  DampingCoefficient=0  DampingCoefficientUnits=N*m/(deg/s)  LowerLimitSpecify=off  LowerLimitBound=-90  LowerLimitBoundUnits=deg  LowerLimitStiffness=1e4  LowerLimitStiffnessUnits=N*m/deg  LowerLimitDamping=10  LowerLimitDampingUnits=N*m/(deg/s)  LowerLimitTransitionRegionWidth=0.1  LowerLimitTransitionRegionWidthUnits=deg  UpperLimitSpecify=off  UpperLimitBound=90  UpperLimitBoundUnits=deg  UpperLimitStiffness=1e4  UpperLimitStiffnessUnits=N*m/deg  UpperLimitDamping=10  UpperLimitDampingUnits=N*m/(deg/s)  UpperLimitTransitionRegionWidth=0.1  UpperLimitTransitionRegionWidthUnits=deg  TorqueActuationMode=NoTorque  MotionActuationMode=ComputedMotion  SensePosition=off  SenseVelocity=off  SenseAcceleration=off  SenseTorqueForce=off  SenseLowerLimitTorqueForce=off  SenseUpperLimitTorqueForce=off
  Revolute Joint1 : sm_lib/Joints/Revolute Joint  JointMode=Normal  CompositeWrenchDir=FollowerOnBase  CompositeWrenchFrame=BaseFrame  SenseConstraintForce=off  SenseConstraintTorque=off  SenseTotalForce=off  SenseTotalTorque=off  PositionTargetSpecify=off  PositionTargetPriority=High  PositionTargetValue=0  PositionTargetValueUnits=deg  VelocityTargetSpecify=off  VelocityTargetPriority=High  VelocityTargetValue=0  VelocityTargetValueUnits=deg/s  EquilibriumPosition=0  EquilibriumPositionUnits=deg  SpringStiffness=0  SpringStiffnessUnits=N*m/deg  DampingCoefficient=0  DampingCoefficientUnits=N*m/(deg/s)  LowerLimitSpecify=off  LowerLimitBound=-90  LowerLimitBoundUnits=deg  LowerLimitStiffness=1e4  LowerLimitStiffnessUnits=N*m/deg  LowerLimitDamping=10  LowerLimitDampingUnits=N*m/(deg/s)  LowerLimitTransitionRegionWidth=0.1  LowerLimitTransitionRegionWidthUnits=deg  UpperLimitSpecify=off  UpperLimitBound=90  UpperLimitBoundUnits=deg  UpperLimitStiffness=1e4  UpperLimitStiffnessUnits=N*m/deg  UpperLimitDamping=10  UpperLimitDampingUnits=N*m/(deg/s)  UpperLimitTransitionRegionWidth=0.1  UpperLimitTransitionRegionWidthUnits=deg  TorqueActuationMode=ComputedTorque  MotionActuationMode=InputMotion  SensePosition=on  SenseVelocity=off  SenseAcceleration=off  SenseTorqueForce=on  SenseLowerLimitTorqueForce=off  SenseUpperLimitTorqueForce=off
  Revolute Joint11 : sm_lib/Joints/Revolute Joint  JointMode=Normal  CompositeWrenchDir=FollowerOnBase  CompositeWrenchFrame=BaseFrame  SenseConstraintForce=off  SenseConstraintTorque=off  SenseTotalForce=off  SenseTotalTorque=off  PositionTargetSpecify=off  PositionTargetPriority=High  PositionTargetValue=-0.919709  PositionTargetValueUnits=deg  VelocityTargetSpecify=off  VelocityTargetPriority=High  VelocityTargetValue=0  VelocityTargetValueUnits=deg/s  EquilibriumPosition=0  EquilibriumPositionUnits=deg  SpringStiffness=0  SpringStiffnessUnits=N*m/deg  DampingCoefficient=0  DampingCoefficientUnits=N*m/(deg/s)  LowerLimitSpecify=off  LowerLimitBound=-90  LowerLimitBoundUnits=deg  LowerLimitStiffness=1e4  LowerLimitStiffnessUnits=N*m/deg  LowerLimitDamping=10  LowerLimitDampingUnits=N*m/(deg/s)  LowerLimitTransitionRegionWidth=0.1  LowerLimitTransitionRegionWidthUnits=deg  UpperLimitSpecify=off  UpperLimitBound=90  UpperLimitBoundUnits=deg  UpperLimitStiffness=1e4  UpperLimitStiffnessUnits=N*m/deg  UpperLimitDamping=10  UpperLimitDampingUnits=N*m/(deg/s)  UpperLimitTransitionRegionWidth=0.1  UpperLimitTransitionRegionWidthUnits=deg  TorqueActuationMode=NoTorque  MotionActuationMode=ComputedMotion  SensePosition=off  SenseVelocity=off  SenseAcceleration=off  SenseTorqueForce=off  SenseLowerLimitTorqueForce=off  SenseUpperLimitTorqueForce=off
  Revolute Joint20 : sm_lib/Joints/Revolute Joint  JointMode=Normal  CompositeWrenchDir=FollowerOnBase  CompositeWrenchFrame=BaseFrame  SenseConstraintForce=off  SenseConstraintTorque=off  SenseTotalForce=off  SenseTotalTorque=off  PositionTargetSpecify=off  PositionTargetPriority=High  PositionTargetValue=40  PositionTargetValueUnits=deg  VelocityTargetSpecify=off  VelocityTargetPriority=High  VelocityTargetValue=0  VelocityTargetValueUnits=deg/s  EquilibriumPosition=0  EquilibriumPositionUnits=deg  SpringStiffness=0  SpringStiffnessUnits=N*m/deg  DampingCoefficient=0  DampingCoefficientUnits=N*m/(deg/s)  LowerLimitSpecify=off  LowerLimitBound=-90  LowerLimitBoundUnits=deg  LowerLimitStiffness=1e4  LowerLimitStiffnessUnits=N*m/deg  LowerLimitDamping=10  LowerLimitDampingUnits=N*m/(deg/s)  LowerLimitTransitionRegionWidth=0.1  LowerLimitTransitionRegionWidthUnits=deg  UpperLimitSpecify=off  UpperLimitBound=90  UpperLimitBoundUnits=deg  UpperLimitStiffness=1e4  UpperLimitStiffnessUnits=N*m/deg  UpperLimitDamping=10  UpperLimitDampingUnits=N*m/(deg/s)  UpperLimitTransitionRegionWidth=0.1  UpperLimitTransitionRegionWidthUnits=deg  TorqueActuationMode=NoTorque  MotionActuationMode=ComputedMotion  SensePosition=off  SenseVelocity=off  SenseAcceleration=off  SenseTorqueForce=off  SenseLowerLimitTorqueForce=off  SenseUpperLimitTorqueForce=off
  Simulink-PS Converter2 : nesl_utility/Simulink-PS Converter  PhysicalDomain=network_engine_domain  SubClassName=ps_input  LeftPortType=input  RightPortType=output  PseudoPeriodic=off  Frequencies=[]  NoiseDistribution=none  NoiseParameters=[]  Unit=rad  AffineConversion=off  FilteringAndDerivatives=filter  SimscapeFilterOrder=2  InputFilterTimeConstant=0.001  UdotUserProvided=0
  Solver Configuration : nesl_utility/Solver Configuration  PhysicalDomain=network_engine_domain  SubClassName=solver  LeftPortType=input  RightPortType=generic  Tones=[]  Harmonics=[]  SimulateNoise=off  Profile=off  UseLocalSampling=off  EnableSwitchedLinearOptims=on  FrequencyDomain=off  UseCCode=off  RelTol=0.001  AbsTol=1e-06  MinStep=1e-09  ToWorkspace=off  RevertToSquareIcSolve=off  NumHomotopyIterations=100  PhasorMode=off  PhasorModeNumHarmonics=1  ConsistencySolver=NEWTON_XTOL_AFTER_FTOL  CanonicalOrdering=UNORDERED  OptimizeIntermediates=UNOPTIMIZED  IndexReductionMethod=DerivativeReplacement  DoDC=off  ResidualTolerance=1e-09  ConsistencyTolSource=GLOBAL  ConsistencyAbsTol=0.001  ConsistencyRelTol=0.001  ConsistencyTolFactor=0.001  UseLocalSolver=off  LocalSolverChoice=NE_BACKWARD_EULER_ADVANCER  ResolveIndetEquations=on  FunctionEvalNumThread=1  LocalSolverSampleTime=0.001  DoFixedCost=off  MaxNonlinIter=3  MaxModeIter=2  ComputeImpulses=off  ImpulseIterations=2  LinearAlgebra=Sparse  LinearAlgebraNumThread=0  EquationFormulation=NE_TIME_EF  DelaysMemoryBudget=1024  AutomaticFiltering=on  FilteringTimeConstant=0.001  PartitionStorageMethod=AS_NEEDED  PartitionMemoryBudget=1024  PartitionMethod=FAST  MultibodyUseLocalSolver=off  MultibodyLocalSolverChoice=ODE1  MultibodyLocalSolverSampleTime=0.001
  To Workspace : ToWorkspace  VariableName=x_wheel  SaveFormat=Timeseries  SampleTime=-1
  To Workspace1 : ToWorkspace  VariableName=v_wheel  SaveFormat=Timeseries  SampleTime=-1
  To Workspace2 : ToWorkspace  VariableName=a_wheel  SaveFormat=Timeseries  SampleTime=-1
  To Workspace3 : ToWorkspace  VariableName=theta_input  SaveFormat=Timeseries  SampleTime=-1
  To Workspace4 : ToWorkspace  VariableName=Torque_input  SaveFormat=Timeseries  SampleTime=-1
  Transform Sensor : sm_lib/Frames and Transforms/Transform Sensor  MeasurementFrame=World  RotationSequence=XYX  SenseAngle=off  SenseAxis=off  SenseQ=off  SenseR=off  SenseRotationSequence=off  SenseOmegaX=off  SenseOmegaY=off  SenseOmegaZ=off  SenseOmega=off  SenseQDot=off  SenseRDot=off  SenseRotationSequenceDot=off  SenseAlphaX=off  SenseAlphaY=off  SenseAlphaZ=off  SenseAlpha=off  SenseQDDot=off  SenseRDDot=off  SenseX=off  SenseY=off  SenseZ=off  SenseXYZ=on  SenseRad=off  SenseAzim=off  SenseDist=off  SenseInc=off  SenseXDot=off  SenseYDot=off  SenseZDot=off  SenseXYZDot=on  SenseRadDot=off  SenseAzimDot=off  SenseDistDot=off  SenseIncDot=off  SenseXDDot=off  SenseYDDot=off  SenseZDDot=off  SenseXYZDDot=on  SenseRadDDot=off  SenseAzimDDot=off  SenseDistDDot=off  SenseIncDDot=off
  Upper piston : sm_lib/Body Elements/File Solid  ExtGeomFileName=C:\Users\USER\Desktop\Term project Machinary\Term-Project-2103322-Design-of-Mechanism_Landing_Gear_Mechanism\simulation\cad\Parts\Upper_Piston1.step  UnitType=FromFile  ExtGeomFileUnits=m  StepReaderType=HEX  ExportConvexHullGeometry=off  InertiaType=CalculateFromGeometry  BasedOnType=Density  Density=1000  DensityUnits=kg/m^3  Mass=1  MassUnits=kg  CenterOfMass=[0 0 0]  CenterOfMassUnits=m  MomentsOfInertia=[1 1 1]  MomentsOfInertiaUnits=kg*m^2  ProductsOfInertia=[0 0 0]  ProductsOfInertiaUnits=kg*m^2  GraphicType=FromGeometry  MarkerShape=Sphere  MarkerSize=10  GraphicVisPropType=FromFileVisualProperties  GraphicDiffuseColor=[0.5 0.5 0.5]  GraphicOpacity=1  GraphicSpecularColor=[0.5 0.5 0.5 1.0]  GraphicAmbientColor=[0.15 0.15 0.15 1.0]  GraphicEmissiveColor=[0.0 0.0 0.0 1.0]  GraphicShininess=75  DoExposeReferenceFrame=off  SerializedFrames=|
      | <Frames>
      | 
      |   <Frame>
      |     <Id>Frame1</Id>
      |     <Value>
      |       <Name>037</Name>
      |       <Origin>
      |         <Source>GeometricFeature</Source>
      |         <FeatureName>circular curve 12</FeatureName>
      |       </Origin>
      |       <PrimaryAxis>
      |         <DefinedDirection>-Z</DefinedDirection>
      |         <Source>GeometricFeature</Source>
      |         <SourceDirection>+Z</SourceDirection>
      |         <FeatureName>circular curve 12</FeatureName>
      |       </PrimaryAxis>
      |       <SecondaryAxis>
      |         <DefinedDirection>+Y</DefinedDirection>
      |         <Source>ReferenceFrame</Source>
      |         <SourceDirection>+Y</SourceDirection>
      |         <FeatureName></FeatureName>
      |       </SecondaryAxis>
      |     </Value>
      |   </Frame>
      | 
      |   <Frame>
      |     <Id>Frame2</Id>
      |     <Value>
      |       <Name>lower</Name>
      |       <Origin>
      |         <Source>GeometricFeature</Source>
      |         <FeatureName>circular curve 48</FeatureName>
      |       </Origin>
      |       <PrimaryAxis>
      |         <DefinedDirection>+Z</DefinedDirection>
      |         <Source>GeometricFeature</Source>
      |         <SourceDirection>+Z</SourceDirection>
      |         <FeatureName>circular curve 48</FeatureName>
      |       </PrimaryAxis>
      |       <SecondaryAxis>
      |         <DefinedDirection>+X</DefinedDirection>
      |         <Source>ReferenceFrame</Source>
      |         <SourceDirection>+X</SourceDirection>
      |         <FeatureName></FeatureName>
      |       </SecondaryAxis>
      |     </Value>
      |   </Frame>
      | 
      | </Frames>
  Weld Joint{,1..3} (4 alike) : sm_lib/Joints/Weld Joint  JointMode=Normal  CompositeWrenchDir=FollowerOnBase  CompositeWrenchFrame=BaseFrame  SenseConstraintForce=off  SenseConstraintTorque=off  SenseTotalForce=off  SenseTotalTorque=off
  Wheel : sm_lib/Body Elements/File Solid  ExtGeomFileName=C:\Users\USER\Desktop\Term project Machinary\Term-Project-2103322-Design-of-Mechanism_Landing_Gear_Mechanism\simulation\cad\Parts\Wheel.step  UnitType=FromFile  ExtGeomFileUnits=m  StepReaderType=HEX  ExportConvexHullGeometry=off  InertiaType=CalculateFromGeometry  BasedOnType=Density  Density=1000  DensityUnits=kg/m^3  Mass=1  MassUnits=kg  CenterOfMass=[0 0 0]  CenterOfMassUnits=m  MomentsOfInertia=[1 1 1]  MomentsOfInertiaUnits=kg*m^2  ProductsOfInertia=[0 0 0]  ProductsOfInertiaUnits=kg*m^2  GraphicType=FromGeometry  MarkerShape=Sphere  MarkerSize=10  GraphicVisPropType=SimpleVisualProperties  GraphicDiffuseColor=[1 0.3333 1]  GraphicOpacity=1  GraphicSpecularColor=[0.5 0.5 0.5 1.0]  GraphicAmbientColor=[0.15 0.15 0.15 1.0]  GraphicEmissiveColor=[0.0 0.0 0.0 1.0]  GraphicShininess=75  DoExposeReferenceFrame=off  SerializedFrames=|
      | <Frames>
      | 
      |   <Frame>
      |     <Id>Frame1</Id>
      |     <Value>
      |       <Name>yellow</Name>
      |       <Origin>
      |         <Source>GeometricFeature</Source>
      |         <FeatureName>circular curve 58</FeatureName>
      |       </Origin>
      |       <PrimaryAxis>
      |         <DefinedDirection>-Z</DefinedDirection>
      |         <Source>GeometricFeature</Source>
      |         <SourceDirection>+Z</SourceDirection>
      |         <FeatureName>circular curve 58</FeatureName>
      |       </PrimaryAxis>
      |       <SecondaryAxis>
      |         <DefinedDirection>+Y</DefinedDirection>
      |         <Source>ReferenceFrame</Source>
      |         <SourceDirection>+Y</SourceDirection>
      |         <FeatureName></FeatureName>
      |       </SecondaryAxis>
      |     </Value>
      |   </Frame>
      | 
      |   <Frame>
      |     <Id>Frame2</Id>
      |     <Value>
      |       <Name>035</Name>
      |       <Origin>
      |         <Source>GeometricFeature</Source>
      |         <FeatureName>circular curve 71</FeatureName>
      |       </Origin>
      |       <PrimaryAxis>
      |         <DefinedDirection>-Z</DefinedDirection>
      |         <Source>GeometricFeature</Source>
      |         <SourceDirection>+Z</SourceDirection>
      |         <FeatureName>circular curve 71</FeatureName>
      |       </PrimaryAxis>
      |       <SecondaryAxis>
      |         <DefinedDirection>+Y</DefinedDirection>
      |         <Source>ReferenceFrame</Source>
      |         <SourceDirection>+Y</SourceDirection>
      |         <FeatureName></FeatureName>
      |       </SecondaryAxis>
      |     </Value>
      |   </Frame>
      | 
      |   <Frame>
      |     <Id>Frame3</Id>
      |     <Value>
      |       <Name>dark g</Name>
      |       <Origin>
      |         <Source>GeometricFeature</Source>
      |         <FeatureName>circular curve 66</FeatureName>
      |       </Origin>
      |       <PrimaryAxis>
      |         <DefinedDirection>-Z</DefinedDirection>
      |         <Source>GeometricFeature</Source>
      |         <SourceDirection>+Z</SourceDirection>
      |         <FeatureName>circular curve 66</FeatureName>
      |       </PrimaryAxis>
      |       <SecondaryAxis>
      |         <DefinedDirection>+Y</DefinedDirection>
      |         <Source>ReferenceFrame</Source>
      |         <SourceDirection>+Y</SourceDirection>
      |         <FeatureName></FeatureName>
      |       </SecondaryAxis>
      |     </Value>
      |   </Frame>
      | 
      |   <Frame>
      |     <Id>Frame4</Id>
      |     <Value>
      |       <Name>purple</Name>
      |       <Origin>
      |         <Source>GeometricFeature</Source>
      |         <FeatureName>circular curve 74</FeatureName>
      |       </Origin>
      |       <PrimaryAxis>
      |         <DefinedDirection>-Z</DefinedDirection>
      |         <Source>GeometricFeature</Source>
      |         <SourceDirection>+Z</SourceDirection>
      |         <FeatureName>circular curve 74</FeatureName>
      |       </PrimaryAxis>
      |       <SecondaryAxis>
      |         <DefinedDirection>+Y</DefinedDirection>
      |         <Source>ReferenceFrame</Source>
      |         <SourceDirection>+Y</SourceDirection>
      |         <FeatureName></FeatureName>
      |       </SecondaryAxis>
      |     </Value>
      |   </Frame>
      | 
      |   <Frame>
      |     <Id>Frame5</Id>
      |     <Value>
      |       <Name>030</Name>
      |       <Origin>
      |         <Source>GeometricFeature</Source>
      |         <FeatureName>circular curve 47</FeatureName>
      |       </Origin>
      |       <PrimaryAxis>
      |         <DefinedDirection>-Z</DefinedDirection>
      |         <Source>GeometricFeature</Source>
      |         <SourceDirection>+Z</SourceDirection>
      |         <FeatureName>circular curve 47</FeatureName>
      |       </PrimaryAxis>
      |       <SecondaryAxis>
      |         <DefinedDirection>+Y</DefinedDirection>
      |         <Source>ReferenceFrame</Source>
      |         <SourceDirection>+Y</SourceDirection>
      |         <FeatureName></FeatureName>
      |       </SecondaryAxis>
      |     </Value>
      |   </Frame>
      | 
      |   <Frame>
      |     <Id>Frame6</Id>
      |     <Value>
      |       <Name>sensor</Name>
      |       <Origin>
      |         <Source>GeometricFeature</Source>
      |         <FeatureName>circular curve 1</FeatureName>
      |       </Origin>
      |       <PrimaryAxis>
      |         <DefinedDirection>+Z</DefinedDirection>
      |         <Source>ReferenceFrame</Source>
      |         <SourceDirection>+Z</SourceDirection>
      |         <FeatureName></FeatureName>
      |       </PrimaryAxis>
      |       <SecondaryAxis>
      |         <DefinedDirection>+X</DefinedDirection>
      |         <Source>ReferenceFrame</Source>
      |         <SourceDirection>+X</SourceDirection>
      |         <FeatureName></FeatureName>
      |       </SecondaryAxis>
      |     </Value>
      |   </Frame>
      | 
      | </Frames>
  World Frame : sm_lib/Frames and Transforms/World Frame
  Yellow : sm_lib/Body Elements/File Solid  ExtGeomFileName=C:\Users\USER\Desktop\Term project Machinary\Term-Project-2103322-Design-of-Mechanism_Landing_Gear_Mechanism\simulation\cad\Parts\Yellow.step  UnitType=FromFile  ExtGeomFileUnits=m  StepReaderType=HEX  ExportConvexHullGeometry=off  InertiaType=CalculateFromGeometry  BasedOnType=Density  Density=1000  DensityUnits=kg/m^3  Mass=1  MassUnits=kg  CenterOfMass=[0 0 0]  CenterOfMassUnits=m  MomentsOfInertia=[1 1 1]  MomentsOfInertiaUnits=kg*m^2  ProductsOfInertia=[0 0 0]  ProductsOfInertiaUnits=kg*m^2  GraphicType=FromGeometry  MarkerShape=Sphere  MarkerSize=10  GraphicVisPropType=FromFileVisualProperties  GraphicDiffuseColor=[0.5 0.5 0.5]  GraphicOpacity=1  GraphicSpecularColor=[0.5 0.5 0.5 1.0]  GraphicAmbientColor=[0.15 0.15 0.15 1.0]  GraphicEmissiveColor=[0.0 0.0 0.0 1.0]  GraphicShininess=75  DoExposeReferenceFrame=off  SerializedFrames=|
      | <Frames>
      | 
      |   <Frame>
      |     <Id>Frame1</Id>
      |     <Value>
      |       <Name>base</Name>
      |       <Origin>
      |         <Source>GeometricFeature</Source>
      |         <FeatureName>circular curve 57</FeatureName>
      |       </Origin>
      |       <PrimaryAxis>
      |         <DefinedDirection>+Z</DefinedDirection>
      |         <Source>GeometricFeature</Source>
      |         <SourceDirection>+Z</SourceDirection>
      |         <FeatureName>circular curve 57</FeatureName>
      |       </PrimaryAxis>
      |       <SecondaryAxis>
      |         <DefinedDirection>+Y</DefinedDirection>
      |         <Source>ReferenceFrame</Source>
      |         <SourceDirection>+Y</SourceDirection>
      |         <FeatureName></FeatureName>
      |       </SecondaryAxis>
      |     </Value>
      |   </Frame>
      | 
      |   <Frame>
      |     <Id>Frame2</Id>
      |     <Value>
      |       <Name>wheel</Name>
      |       <Origin>
      |         <Source>GeometricFeature</Source>
      |         <FeatureName>circular curve 45</FeatureName>
      |       </Origin>
      |       <PrimaryAxis>
      |         <DefinedDirection>+Z</DefinedDirection>
      |         <Source>GeometricFeature</Source>
      |         <SourceDirection>+Z</SourceDirection>
      |         <FeatureName>circular curve 45</FeatureName>
      |       </PrimaryAxis>
      |       <SecondaryAxis>
      |         <DefinedDirection>+Y</DefinedDirection>
      |         <Source>ReferenceFrame</Source>
      |         <SourceDirection>+Y</SourceDirection>
      |         <FeatureName></FeatureName>
      |       </SecondaryAxis>
      |     </Value>
      |   </Frame>
      | 
      | </Frames>
  light green1 : sm_lib/Body Elements/File Solid  ExtGeomFileName=C:\Users\USER\Desktop\Term project Machinary\Term-Project-2103322-Design-of-Mechanism_Landing_Gear_Mechanism\simulation\cad\Parts\extragreen.step  UnitType=FromFile  ExtGeomFileUnits=m  StepReaderType=HEX  ExportConvexHullGeometry=off  InertiaType=CalculateFromGeometry  BasedOnType=Density  Density=1000  DensityUnits=kg/m^3  Mass=1  MassUnits=kg  CenterOfMass=[0 0 0]  CenterOfMassUnits=m  MomentsOfInertia=[1 1 1]  MomentsOfInertiaUnits=kg*m^2  ProductsOfInertia=[0 0 0]  ProductsOfInertiaUnits=kg*m^2  GraphicType=FromGeometry  MarkerShape=Sphere  MarkerSize=10  GraphicVisPropType=SimpleVisualProperties  GraphicDiffuseColor=[0.2902 1 0.3961]  GraphicOpacity=1  GraphicSpecularColor=[0.5 0.5 0.5 1.0]  GraphicAmbientColor=[0.15 0.15 0.15 1.0]  GraphicEmissiveColor=[0.0 0.0 0.0 1.0]  GraphicShininess=75  DoExposeReferenceFrame=off  SerializedFrames=|
      | <Frames>
      | 
      |   <Frame>
      |     <Id>Frame1</Id>
      |     <Value>
      |       <Name>036</Name>
      |       <Origin>
      |         <Source>GeometricFeature</Source>
      |         <FeatureName>cylindrical surface 18</FeatureName>
      |       </Origin>
      |       <PrimaryAxis>
      |         <DefinedDirection>+Z</DefinedDirection>
      |         <Source>GeometricFeature</Source>
      |         <SourceDirection>+Z</SourceDirection>
      |         <FeatureName>cylindrical surface 18</FeatureName>
      |       </PrimaryAxis>
      |       <SecondaryAxis>
      |         <DefinedDirection>+Y</DefinedDirection>
      |         <Source>ReferenceFrame</Source>
      |         <SourceDirection>+Y</SourceDirection>
      |         <FeatureName></FeatureName>
      |       </SecondaryAxis>
      |     </Value>
      |   </Frame>
      | 
      |   <Frame>
      |     <Id>Frame2</Id>
      |     <Value>
      |       <Name>037</Name>
      |       <Origin>
      |         <Source>GeometricFeature</Source>
      |         <FeatureName>circular curve 14</FeatureName>
      |       </Origin>
      |       <PrimaryAxis>
      |         <DefinedDirection>+Z</DefinedDirection>
      |         <Source>GeometricFeature</Source>
      |         <SourceDirection>+Z</SourceDirection>
      |         <FeatureName>circular curve 14</FeatureName>
      |       </PrimaryAxis>
      |       <SecondaryAxis>
      |         <DefinedDirection>+Y</DefinedDirection>
      |         <Source>ReferenceFrame</Source>
      |         <SourceDirection>+Y</SourceDirection>
      |         <FeatureName></FeatureName>
      |       </SecondaryAxis>
      |     </Value>
      |   </Frame>
      | 
      |   <Frame>
      |     <Id>Frame3</Id>
      |     <Value>
      |       <Name>red</Name>
      |       <Origin>
      |         <Source>GeometricFeature</Source>
      |         <FeatureName>circular curve 52</FeatureName>
      |       </Origin>
      |       <PrimaryAxis>
      |         <DefinedDirection>+Z</DefinedDirection>
      |         <Source>GeometricFeature</Source>
      |         <SourceDirection>+Z</SourceDirection>
      |         <FeatureName>circular curve 52</FeatureName>
      |       </PrimaryAxis>
      |       <SecondaryAxis>
      |         <DefinedDirection>+X</DefinedDirection>
      |         <Source>ReferenceFrame</Source>
      |         <SourceDirection>+X</SourceDirection>
      |         <FeatureName></FeatureName>
      |       </SecondaryAxis>
      |     </Value>
      |   </Frame>
      | 
      | </Frames>
  wires:
  PS-Simulink Converter1/1 -> Display1/1  "x(mm)"
  Repeating Sequence1/1 -> Simulink-PS Converter2/1
  PS-Simulink Converter2/1 -> Display2/1  "v(mm/s)"
  PS-Simulink Converter3/1 -> Display3/1  "a(mm/s^2)"
  PS-Simulink Converter4/1 -> To Workspace4/1, Display4/1  "Torque(N.m)"
  PS-Simulink Converter7/1 -> To Workspace2/1, Display7/1  "a_wheel(mm/s^2) (x,y,z)"
  PS-Simulink Converter5/1 -> To Workspace/1, Display5/1  "x_wheel(mm) (x,y,z)"
  PS-Simulink Converter6/1 -> To Workspace1/1, Display6/1  "v_wheel(mm/s) (x,y,z)"
  PS-Simulink Converter8/1 -> To Workspace3/1, Display8/1  "theta(deg)"
  connections:
  World Frame/RConn1 -- Mechanism Configuration/RConn1 -- Transform Sensor/LConn1 -- Solver Configuration/RConn1 -- Base/RConn1
  Base/RConn2 -- Revolute Joint2/LConn1
  Base/LConn1 -- Revolute Joint/LConn1
  Base/LConn2 -- Revolute Joint1/LConn1
  Revolute Joint2/RConn1 -- 036/LConn1
  Revolute Joint1/RConn1 -- 032_2/LConn1
  036/RConn1 -- Weld Joint/LConn1
  light green1/RConn1 -- 037/LConn1
  037/RConn1 -- Revolute Joint3/LConn1
  Upper piston/LConn1 -- Revolute Joint3/RConn1
  Prismatic Joint/LConn1 -- Upper piston/RConn1
  Prismatic Joint/RConn1 -- Lower piston/LConn1
  032_2/RConn1 -- Weld Joint1/LConn1
  Revolute Joint20/RConn1 -- Lower piston/RConn1
  Orange/LConn1 -- Weld Joint2/LConn1
  031/LConn1 -- Weld Joint2/RConn1
  Purple/LConn2 -- Revolute Joint19/LConn1
  Revolute Joint11/RConn1 -- Yellow/LConn1
  Revolute Joint11/LConn1 -- Base/LConn3
  Weld Joint3/LConn1 -- light green1/LConn2
  Revolute Joint15/LConn1 -- Yellow/RConn1
  Revolute Joint15/RConn1 -- Wheel/LConn1
  Wheel/RConn1 -- 035/LConn1
  Revolute Joint7/LConn1 -- Wheel/LConn2
  Revolute Joint7/RConn1 -- Dark green/LConn1
  Wheel/RConn2 -- Revolute Joint14/RConn1
  Revolute Joint17/RConn1 -- 030/LConn1
  Revolute Joint17/LConn1 -- Wheel/LConn3
  034/RConn1 -- Weld Joint3/RConn1
  Purple/LConn3 -- 041/LConn1
  Weld Joint/RConn1 -- light green1/LConn1
  Revolute Joint5/LConn1 -- 033/LConn1
  Revolute Joint6/LConn1 -- 033/RConn1
  Revolute Joint5/RConn1 -- Orange/RConn1
  Red/LConn1 -- Revolute Joint6/RConn1
  034/LConn1 -- Red/RConn1
  Purple/RConn2 -- Revolute Joint14/LConn1
  031/RConn1 -- Revolute Joint19/RConn1
  Weld Joint1/RConn1 -- Purple/LConn1
  Purple/RConn1 -- Revolute Joint20/LConn1
  Dark green/RConn1 -- Revolute Joint4/LConn1
  Revolute Joint/RConn1 -- 302_3/LConn1
  Revolute Joint4/RConn1 -- 302_3/RConn1
  Prismatic Joint/RConn2 -- PS-Simulink Converter1/LConn1
  Simulink-PS Converter2/RConn1 -- Revolute Joint1/LConn2
  PS-Simulink Converter2/LConn1 -- Prismatic Joint/RConn3
  PS-Simulink Converter3/LConn1 -- Prismatic Joint/RConn4
  PS-Simulink Converter4/LConn1 -- Revolute Joint1/RConn3
  Transform Sensor/RConn1 -- Wheel/RConn3
  PS-Simulink Converter6/LConn1 -- Transform Sensor/RConn3
  PS-Simulink Converter5/LConn1 -- Transform Sensor/RConn2
  PS-Simulink Converter7/LConn1 -- Transform Sensor/RConn4
  PS-Simulink Converter8/LConn1 -- Revolute Joint1/RConn2
